simulink model "perception_simulator"  (R2026a)
settings: Solver=VariableStepAuto  StopTime=60
undefined symbols (not defined in the file or in its folder): Sim3dSensor
libraries: simulink x1, sim3dcameralib x1, sim3dphyssensorlib x1, sim3dlib x1, sim3dautolib x1
settings Model: Creator=jys1n22  LastModifiedBy=jys1n22

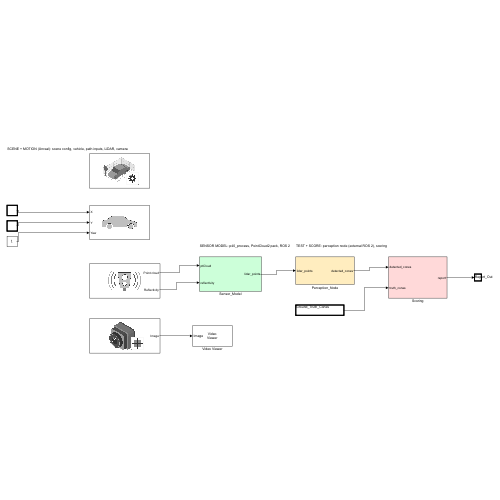
[thumbnail: Simulink's stored preview of the top-level diagram]
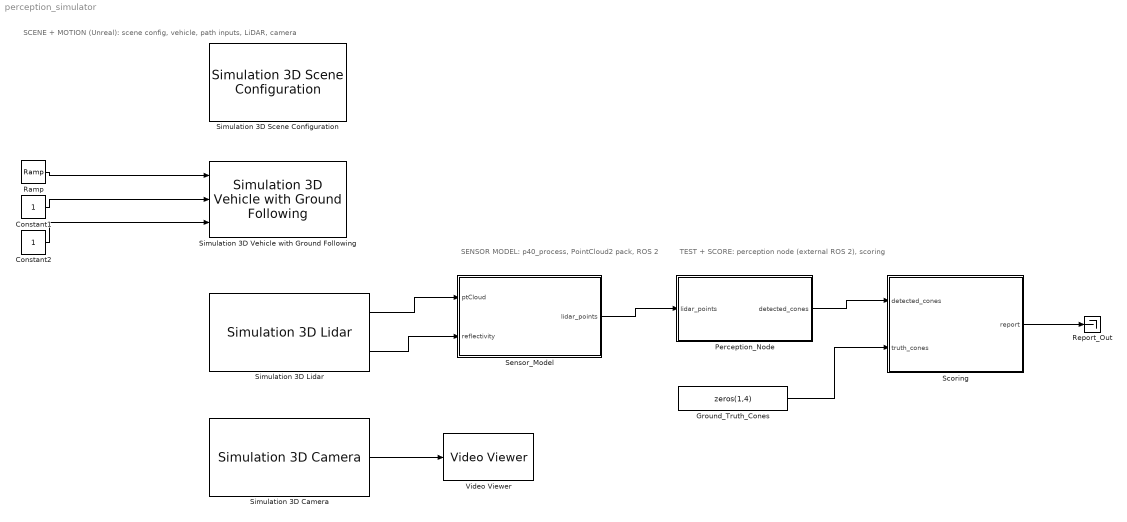
== system perception_simulator ==
  note: SCENE + MOTION (Unreal): scene config, vehicle, path inputs, LiDAR, camera
  note: SENSOR MODEL: p40_process, PointCloud2 pack, ROS 2
  note: TEST + SCORE: perception node (external ROS 2), scoring
  Constant1 : Constant
  Constant2 : Constant
  Ground_Truth_Cones : Constant  Value=zeros(1,4)
  Perception_Node : Subsystem
  Ramp : simulink/Sources/Ramp  slope=5  start=0  InitialOutput=0
  Report_Out : Terminator
  Scoring : Subsystem
  Sensor_Model : Subsystem
  Simulation 3D Camera : sim3dcameralib/Simulation 3D Camera  Priority=2  sensorTag=Sim3dSensor�  sensorId=3  sensorName=Sim3dSensor�  vehTagList={'Custom ...';'Scene Origin';'SimulinkVehicle1'}  vehTag=SimulinkVehicle1  CoordinateSystem=ISO8855  mountLoc=Roof center  offsetFlag=off  tmountOffset=[0, 1.5, 0]  extTmount=off  rmountOffset=[0, 0, 0]  extRmount=off  FocalLength=[1109, 1109]  OpticalCenter=[640, 360]  ImageSize=[720, 1280]  RadialDistortion=[0, 0]  TangentialDistortion=[0, 0]  SensorSkew=0  VisualizeFieldOfView=off  FieldOfViewRange=61  DepthOutportEnabled=off  SemanticOutportEnabled=off  TransformOutportEnabled=off  SampleTime=0.1  mountPoint=[-0.25 0 1.57]  mountOrientation=[0 0 0]  aMode=3  ID=3
      settings: LibrarySourceBlock=drivingsim3d/Simulation 3D Camera
  Simulation 3D Lidar : sim3dphyssensorlib/Simulation 3D Lidar  Priority=2  sensorTag=Sim3dSensor�  sensorId=2  sensorName=Sim3dSensor�  vehTagList={'Custom ...';'Scene Origin';'SimulinkVehicle1'}  vehTag=SimulinkVehicle1  CoordinateSystem=ISO8855  mountLoc=Roof center  offsetFlag=off  tmountOffset=[0, 1.5, 0]  rmountOffset=[0, 0, 0]  DetectionRange=200  RangeResolution=0.004  FieldOfViewSpecification=Asymmetric  VerticalFOV=40  VerticalFOVBounds=single([-25 15])  VerticalResolution=1/3  VerticalSampleAngles=-20:20  HorizontalFOV=360  HorizontalFOVBounds=single([-180 180])  HorizontalResolution=0.2  HorizontalSampleAngles=-180:180  DistanceOutportEnabled=off  ReflectivityOutportEnabled=on  SemanticOutportEnabled=off  TransformOutportEnabled=off  SampleTime=0.1  mountPoint=[0 0 0]  mountOrientation=[0 0 0]  aMode=3  ID=2
      settings: LibrarySourceBlock=drivingsim3d/Simulation 3D Lidar
  Simulation 3D Scene Configuration : sim3dlib/Simulation 3D Scene Configuration  Priority=0  ProjectFormat=Default Scenes  SceneDesc=US city block  ProjectName=C:\Program Files\MATLAB\2026a\toolbox\shared\sim3d_projects\automotive_project_windows\UE\WindowsNoEditor\VehicleSimulation.exe  ScenePath=/Game/Maps/HwStrght  EnableOpenDRIVE=off  vehTagList={'Custom';'Scene Origin';'SimulinkVehicle1'}  vehTag=Scene Origin  AttachedCameraRelativeTranslation=[0 0 0]  FreeCameraDefaultInitialTranslation=[-6, 0, 2]  AttachedCameraRelativeRotation=[0, -15, 0]  FreeCameraDefaultInitialRotation=[0, -15, 0]  ViewpointName=Custom  FreeCameraInitialTranslation=[0, 0, 0]  FreeCameraInitialRotation=[0, 0, 0]  OpVisEn=off  Ts=0.01  EnableWindow=on  EnableRemoteAccess=off  SimulationMode=CoSimulation  SimulateUsing=Interpreted execution  EnableAnimationRecording=off  OverrideDefaultRecording=off  AnimationRecordingFileName=sim3dAnimation.mat  AnimationRecordingInterval=[0 inf]  EnableWeather=off  SunAzimuth=90  SunAltitude=40.0  EnableGeospatialSun=off  Latitude=0  Longitude=0  Date=2023-01-01  Time=10:30:00  GeoTimeZone=-5.0  SunDaylightSaving=off  wind=1  clouds=10  EnableVolumetricClouds=off  CloudCoverage=0  CloudAltitude=6  fog=0  rain=0  RaindropsEffect=off  SnowDensity=0  EnableGeospatial=off  TilesetSource=Earth terrain  UseTrueOrigin=off  OriginHeight=200  OriginLatitude=40.744652  OriginLongitude=-73.988864  MapStyle=Aerial  AdditionalAssetIDs=[]  UseAdvancedSunSky=off  SolarTime=11  TimeZone=-5  Day=21  Month=9  Year=2022  UseDaylightSavingTime=on  DSTStartDay=10  DSTStartMonth=3  DSTEndDay=3  DSTEndMonth=11  DSTSwitchHour=2  sensorTag=MainCamera1  sensorId=1  sensorName=MainCamera1  mountLoc=Origin  offsetFlag=off  tmountOffset=[0, 0, 0]  rmountOffset=[0, 0, 0]  HorizontalResolution=1280  VerticalResolution=720  HorizontalFOV=60  mountPoint=[0 0 0]  mountOrientation=[0 0 0]  aMode=3  ID=1  GeoTrigger=Inactive  ViewNameList={'Custom'}  ViewTranslationList={'[0 0 0]'}  ViewRotationList={'[0 0 0]'}
      settings: LibrarySourceBlock=drivingsim3d/Simulation 3D Scene Configuration
  Simulation 3D Vehicle with Ground Following : sim3dautolib/Simulation 3D Vehicle with Ground Following  Priority=1  PassVehMesh=Muscle car  MeshPath=/MathWorksAutomotiveContent/Vehicles/Muscle/Meshes/SK_MuscleCar.SK_MuscleCar  TrackWidth=1.9  WheelBase=3  WheelRadius=0.35  VehColor=Blue  CoordinateSystem=ISO8855  InitialPos=[0, 0, 0]  InitialRot=[0, 0, 0]  ActorName=SimulinkVehicle1  SampleTime=0.01  ActorType=SimulinkVehicle  ID=1  aMode=3  ActorTag=SimulinkVehicle1  CoordinateScheme=0  VehLightsControl=off  HeadlightColor=[ 1, 1, 1 ]  HighBeamIntensity=100000  LowBeamIntensity=60000  HighBeamConeAngle=70  LowBeamConeAngle=70  LeftHeadlightOrientation=[ 0, 0 ]  RightHeadlightOrientation=[ 0, 0 ]  BrakelightIntensity=500  ReverselightIntensity=500  SignallightIntensity=500  SignallightPeriod=1  SignalPulseWidth=50  TransformOutportEnabled=off
      settings: LibrarySourceBlock=drivingsim3d/Simulation 3D Vehicle with Ground Following
  Video Viewer : VideoViewer  FigPos=[79 1503 1177 920]
  wires:
  Ramp/1 -> Simulation 3D Vehicle with Ground Following/1
  Constant1/1 -> Simulation 3D Vehicle with Ground Following/2
  Constant2/1 -> Simulation 3D Vehicle with Ground Following/3
  Simulation 3D Camera/1 -> Video Viewer/1
  Simulation 3D Lidar/2 -> Sensor_Model/2(reflectivity)
  Sensor_Model/1(lidar_points) -> Perception_Node/1(lidar_points)
  Perception_Node/1(detected_cones) -> Scoring/1(detected_cones)
  Ground_Truth_Cones/1 -> Scoring/2(truth_cones)
  Scoring/1(report) -> Report_Out/1
  Simulation 3D Lidar/1 -> Sensor_Model/1(ptCloud)

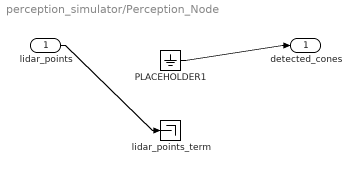
== system perception_simulator/Perception_Node ==
  lidar_points : Inport
  PLACEHOLDER1 : Ground
  lidar_points_term : Terminator
  detected_cones : Outport
  wires:
  lidar_points/1 -> lidar_points_term/1
  PLACEHOLDER1/1 -> detected_cones/1

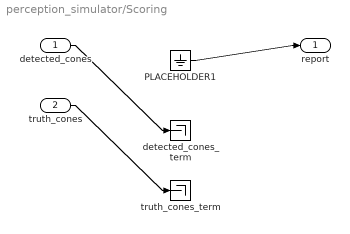
== system perception_simulator/Scoring ==
  detected_cones : Inport
  truth_cones : Inport  Port=2
  PLACEHOLDER1 : Ground
  detected_cones_term : Terminator
  truth_cones_term : Terminator
  report : Outport
  wires:
  detected_cones/1 -> detected_cones_term/1
  truth_cones/1 -> truth_cones_term/1
  PLACEHOLDER1/1 -> report/1

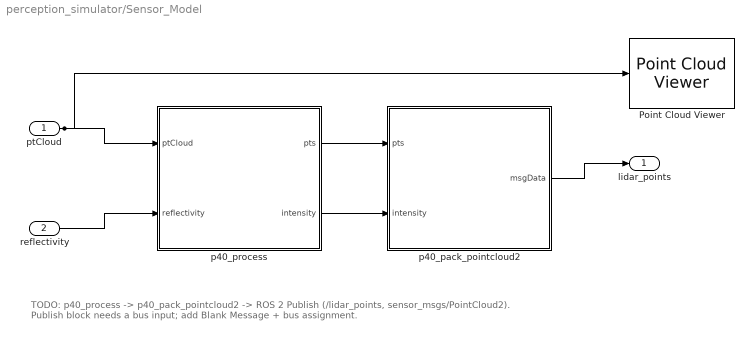
== system perception_simulator/Sensor_Model ==
  note: TODO: p40_process -> p40_pack_pointcloud2 -> ROS 2 Publish (/lidar_points, sensor_msgs/PointCloud2). Publish block needs a bus input; add Blank Message + bus assignment.
  ptCloud : Inport
  reflectivity : Inport  Port=2
  Point Cloud Viewer : PointCloudViewer  FigPos=[1282 1389 1278 1311]  FigSettingsValue=[-40 40 -40 40 -3 5 1]
  p40_pack_pointcloud2 : MATLAB Function  TreatAsAtomicUnit=on
  p40_process : MATLAB Function  TreatAsAtomicUnit=on
  lidar_points : Outport
  wires:
  ptCloud/1 -> Point Cloud Viewer/1, p40_process/1(ptCloud)
  reflectivity/1 -> p40_process/2(reflectivity)
  p40_process/1(pts) -> p40_pack_pointcloud2/1(pts)
  p40_process/2(intensity) -> p40_pack_pointcloud2/2(intensity)
  p40_pack_pointcloud2/1(msgData) -> lidar_points/1

== matlab function perception_simulator/Sensor_Model/p40_process ==
  data: ptCloud input; pts output; reflectivity input; intensity output
function [pts, intensity] = p40_process(ptCloud, reflectivity)
% PLACEHOLDER: keep 40 Pandar40P rows (P40.rowIdx), add range noise,
% dropout, range limits, ISO8855 -> Hesai frame (x_h=-y, y_h=x, z_h=z).
pts = ptCloud;
intensity = reflectivity;
end

== matlab function perception_simulator/Sensor_Model/p40_pack_pointcloud2 ==
  data: pts input; msgData output; intensity input
function msgData = p40_pack_pointcloud2(pts, intensity) %#ok<INUSD>
% PLACEHOLDER: pack x,y,z,intensity (float32) + ring (uint16), 18 B/point.
msgData = zeros(72000*18, 1, 'uint8');
end
